simulink model "IEEE33_TR_TEMPORAL_RECOGNIZABILITY_MASTER"  (R2026b)
settings: Solver=ode23t  StopTime=0.2  MaxStep=1e-5
undefined symbols (not defined in the file): Three_PhaseBreaker_class, Three_PhaseSeriesRLCLoad_class, Three_PhaseSource_class, Three_PhaseV_IMeasuremen_class
libraries: ee_lib x146, nesl_utility x106, fl_lib x33, eeRmsMeasurement x2
(part 4 of 7)

== system IEEE33_TR_TEMPORAL_RECOGNIZABILITY_MASTER/Bus_15/Bus_15 ==
  Current and Voltage Sensor (Three-Phase) : ee_lib/Sensors & Transducers/Current and Voltage Sensor (Three-Phase)  port_option=ee.enum.threePhasePort.expanded  vMeasurementType=1  outputUnit=2  SRated=100000000 V*A  VRated=500000 V  I_specify=off  I_priority=None  I=[ 0 0 0 ] A  I_nominal_specify=off  I_nominal_value=1  I_nominal_unit=A  V_specify=off  V_priority=None  V=[ 0 0 0 ] V  V_nominal_specify=off  V_nominal_value=1  V_nominal_unit=V
  Igain : Gain  Gain=Three_PhaseV_IMeasuremen_class('phase-to-phase','yes','off','off','off',100000000,500000).objParamMappingDerived.NewDerivedParam.IG
  PS-Simulink Converter : nesl_utility/PS-Simulink Converter  PhysicalDomain=network_engine_domain  SubClassName=ps_output  LeftPortType=input  RightPortType=output  PseudoPeriodic=off  Frequencies=[]  VectorFormat=1-D array  Unit=1  AffineConversion=off
  PS-Simulink Converter1 : nesl_utility/PS-Simulink Converter  PhysicalDomain=network_engine_domain  SubClassName=ps_output  LeftPortType=input  RightPortType=output  PseudoPeriodic=off  Frequencies=[]  VectorFormat=1-D array  Unit=1  AffineConversion=off
  Vgain : Gain  Gain=Three_PhaseV_IMeasuremen_class('phase-to-phase','yes','off','off','off',100000000,500000).objParamMappingDerived.NewDerivedParam.VG
  A : PMIOPort  Side=Left
  B : PMIOPort  Port=2  Side=Left
  C : PMIOPort  Port=3  Side=Left
  a : PMIOPort  Port=4  Side=Right
  b : PMIOPort  Port=5  Side=Right
  c : PMIOPort  Port=6  Side=Right
  Vabc : Outport  VectorParamsAs1DForOutWhenUnconnected=off
  Iabc : Outport  Port=2  VectorParamsAs1DForOutWhenUnconnected=off
  wires:
  Igain/1 -> Iabc/1
  Vgain/1 -> Vabc/1
  PS-Simulink Converter1/1 -> Igain/1
  PS-Simulink Converter/1 -> Vgain/1
  connections:
  Current and Voltage Sensor (Three-Phase)/RConn1 -- PS-Simulink Converter/LConn1
  Current and Voltage Sensor (Three-Phase)/RConn2 -- PS-Simulink Converter1/LConn1
  Current and Voltage Sensor (Three-Phase)/RConn5 -- c/RConn1
  Current and Voltage Sensor (Three-Phase)/RConn4 -- b/RConn1
  Current and Voltage Sensor (Three-Phase)/RConn3 -- a/RConn1
  Current and Voltage Sensor (Three-Phase)/LConn3 -- C/RConn1
  Current and Voltage Sensor (Three-Phase)/LConn1 -- A/RConn1
  Current and Voltage Sensor (Three-Phase)/LConn2 -- B/RConn1

== system IEEE33_TR_TEMPORAL_RECOGNIZABILITY_MASTER/Bus_15/CB3-2 ==
  com : Inport
  Add : Sum
  Circuit Breaker : ee_lib/Switches & Breakers/Circuit Breaker (Three-Phase)  port_option=ee.enum.threePhasePort.expanded  control_port_option=ee.enum.controlport.ps  R_closed=0.01 Ohm  G_open=Three_PhaseBreaker_class('open',1000000,Inf,[0.0166666666666667 0.0833333333333333],'on').objParamMappingDerived.NewDerivedParam.G_open 1/Ohm  threshold=0.5 V  breaker_behavior=ee.enum.switches.breakerBehavior.zeroCrossingEnable  i_th=1e-8 A
  Data Type Conversion : DataTypeConversion  OutDataTypeStr=double  SaturateOnIntegerOverflow=off  RndMeth=Floor
  NOT : Logic  Operator=NOT  IconShape=distinctive  AllPortsSameDT=off  OutDataTypeStr=boolean
  Simulink-PS Converter : nesl_utility/Simulink-PS Converter  PhysicalDomain=network_engine_domain  SubClassName=ps_input  LeftPortType=input  RightPortType=output  PseudoPeriodic=off  Frequencies=[]  NoiseDistribution=none  NoiseParameters=[]  Unit=1  AffineConversion=off  FilteringAndDerivatives=provide  SimscapeFilterOrder=1  InputFilterTimeConstant=0.001  UdotUserProvided=0
  Step : Step  Time=1e-6  InitialValue=Three_PhaseBreaker_class('open',1000000,Inf,[0.0166666666666667 0.0833333333333333],'on').objParamMappingDerived.NewDerivedParam.StepInitialValue  FinalValue=0  SampleTime=0
  A : PMIOPort  Side=Left
  B : PMIOPort  Port=2  Side=Left
  C : PMIOPort  Port=3  Side=Left
  a : PMIOPort  Port=4  Side=Right
  b : PMIOPort  Port=5  Side=Right
  c : PMIOPort  Port=6  Side=Right
  wires:
  com/1 -> Add/1
  Add/1 -> NOT/1
  Step/1 -> Add/2
  Data Type Conversion/1 -> Simulink-PS Converter/1
  NOT/1 -> Data Type Conversion/1
  connections:
  Circuit Breaker/LConn1 -- Simulink-PS Converter/RConn1
  c/RConn1 -- Circuit Breaker/RConn3
  b/RConn1 -- Circuit Breaker/RConn2
  a/RConn1 -- Circuit Breaker/RConn1
  Circuit Breaker/LConn4 -- C/RConn1
  Circuit Breaker/LConn3 -- B/RConn1
  Circuit Breaker/LConn2 -- A/RConn1

== system IEEE33_TR_TEMPORAL_RECOGNIZABILITY_MASTER/Bus_15/VI Recorder18 ==
  Vrec : Inport
  Irec : Inport  Port=2
  tag scope: I14to15=global, V14to15=global
  wires:
  Vrec/1 -> [V14to15]
  Irec/1 -> [I14to15]

== system IEEE33_TR_TEMPORAL_RECOGNIZABILITY_MASTER/Bus_16/Bus Load 16 ==
  Electrical Reference : fl_lib/Electrical/Electrical Elements/Electrical Reference
  Wye-Connected Load : ee_lib/Passive/RLC Assemblies/Wye-Connected Load  port_option=ee.enum.threePhasePort.expanded  parameterization=2  component_structure=4  component_structure_PQ=4  R=1 Ohm  L=0.001 H  C=1e-6 F  VRated=11594.6483 V  FRated=60 Hz  P=60000 W  Qpos=20000 V*A  Qneg=Three_PhaseSeriesRLCLoad_class(0).objParamMappingDerived.NewDerivedParam.Qneg V*A  R_parasitic=1e-6 Ohm  G_parasitic=1e-6 1/Ohm  R_parasitic_PQ=1e-6 Ohm  G_parasitic_PQ=1e-6 1/Ohm  Vmag0=11594.6483 V  Vang0=0 deg  Freq0=60 Hz  IL_specify=on  IL_priority=High  IL=[ 0 0 0 ] A  IL_nominal_specify=off  IL_nominal_value=1  IL_nominal_unit=A  VC_specify=on  VC_priority=High  VC=[ 0 0 0 ] V  VC_nominal_specify=off  VC_nominal_value=1  VC_nominal_unit=V
  A : PMIOPort  Side=Left
  B : PMIOPort  Port=2  Side=Left
  C : PMIOPort  Port=3  Side=Left
  connections:
  Electrical Reference/LConn1 -- Wye-Connected Load/RConn1
  Wye-Connected Load/LConn3 -- C/RConn1
  Wye-Connected Load/LConn1 -- A/RConn1
  Wye-Connected Load/LConn2 -- B/RConn1

== system IEEE33_TR_TEMPORAL_RECOGNIZABILITY_MASTER/Bus_16/Bus_16 ==
  Current and Voltage Sensor (Three-Phase) : ee_lib/Sensors & Transducers/Current and Voltage Sensor (Three-Phase)  port_option=ee.enum.threePhasePort.expanded  vMeasurementType=1  outputUnit=2  SRated=100000000 V*A  VRated=500000 V  I_specify=off  I_priority=None  I=[ 0 0 0 ] A  I_nominal_specify=off  I_nominal_value=1  I_nominal_unit=A  V_specify=off  V_priority=None  V=[ 0 0 0 ] V  V_nominal_specify=off  V_nominal_value=1  V_nominal_unit=V
  Igain : Gain  Gain=Three_PhaseV_IMeasuremen_class('phase-to-phase','yes','off','off','off',100000000,500000).objParamMappingDerived.NewDerivedParam.IG
  PS-Simulink Converter : nesl_utility/PS-Simulink Converter  PhysicalDomain=network_engine_domain  SubClassName=ps_output  LeftPortType=input  RightPortType=output  PseudoPeriodic=off  Frequencies=[]  VectorFormat=1-D array  Unit=1  AffineConversion=off
  PS-Simulink Converter1 : nesl_utility/PS-Simulink Converter  PhysicalDomain=network_engine_domain  SubClassName=ps_output  LeftPortType=input  RightPortType=output  PseudoPeriodic=off  Frequencies=[]  VectorFormat=1-D array  Unit=1  AffineConversion=off
  Vgain : Gain  Gain=Three_PhaseV_IMeasuremen_class('phase-to-phase','yes','off','off','off',100000000,500000).objParamMappingDerived.NewDerivedParam.VG
  A : PMIOPort  Side=Left
  B : PMIOPort  Port=2  Side=Left
  C : PMIOPort  Port=3  Side=Left
  a : PMIOPort  Port=4  Side=Right
  b : PMIOPort  Port=5  Side=Right
  c : PMIOPort  Port=6  Side=Right
  Vabc : Outport  VectorParamsAs1DForOutWhenUnconnected=off
  Iabc : Outport  Port=2  VectorParamsAs1DForOutWhenUnconnected=off
  wires:
  Igain/1 -> Iabc/1
  Vgain/1 -> Vabc/1
  PS-Simulink Converter1/1 -> Igain/1
  PS-Simulink Converter/1 -> Vgain/1
  connections:
  Current and Voltage Sensor (Three-Phase)/RConn1 -- PS-Simulink Converter/LConn1
  Current and Voltage Sensor (Three-Phase)/RConn2 -- PS-Simulink Converter1/LConn1
  Current and Voltage Sensor (Three-Phase)/RConn5 -- c/RConn1
  Current and Voltage Sensor (Three-Phase)/RConn4 -- b/RConn1
  Current and Voltage Sensor (Three-Phase)/RConn3 -- a/RConn1
  Current and Voltage Sensor (Three-Phase)/LConn3 -- C/RConn1
  Current and Voltage Sensor (Three-Phase)/LConn1 -- A/RConn1
  Current and Voltage Sensor (Three-Phase)/LConn2 -- B/RConn1

== system IEEE33_TR_TEMPORAL_RECOGNIZABILITY_MASTER/Bus_16/CB3-2 ==
  com : Inport
  Add : Sum
  Circuit Breaker : ee_lib/Switches & Breakers/Circuit Breaker (Three-Phase)  port_option=ee.enum.threePhasePort.expanded  control_port_option=ee.enum.controlport.ps  R_closed=0.01 Ohm  G_open=Three_PhaseBreaker_class('open',1000000,Inf,[0.0166666666666667 0.0833333333333333],'on').objParamMappingDerived.NewDerivedParam.G_open 1/Ohm  threshold=0.5 V  breaker_behavior=ee.enum.switches.breakerBehavior.zeroCrossingEnable  i_th=1e-8 A
  Data Type Conversion : DataTypeConversion  OutDataTypeStr=double  SaturateOnIntegerOverflow=off  RndMeth=Floor
  NOT : Logic  Operator=NOT  IconShape=distinctive  AllPortsSameDT=off  OutDataTypeStr=boolean
  Simulink-PS Converter : nesl_utility/Simulink-PS Converter  PhysicalDomain=network_engine_domain  SubClassName=ps_input  LeftPortType=input  RightPortType=output  PseudoPeriodic=off  Frequencies=[]  NoiseDistribution=none  NoiseParameters=[]  Unit=1  AffineConversion=off  FilteringAndDerivatives=provide  SimscapeFilterOrder=1  InputFilterTimeConstant=0.001  UdotUserProvided=0
  Step : Step  Time=1e-6  InitialValue=Three_PhaseBreaker_class('open',1000000,Inf,[0.0166666666666667 0.0833333333333333],'on').objParamMappingDerived.NewDerivedParam.StepInitialValue  FinalValue=0  SampleTime=0
  A : PMIOPort  Side=Left
  B : PMIOPort  Port=2  Side=Left
  C : PMIOPort  Port=3  Side=Left
  a : PMIOPort  Port=4  Side=Right
  b : PMIOPort  Port=5  Side=Right
  c : PMIOPort  Port=6  Side=Right
  wires:
  com/1 -> Add/1
  Add/1 -> NOT/1
  Step/1 -> Add/2
  Data Type Conversion/1 -> Simulink-PS Converter/1
  NOT/1 -> Data Type Conversion/1
  connections:
  Circuit Breaker/LConn1 -- Simulink-PS Converter/RConn1
  c/RConn1 -- Circuit Breaker/RConn3
  b/RConn1 -- Circuit Breaker/RConn2
  a/RConn1 -- Circuit Breaker/RConn1
  Circuit Breaker/LConn4 -- C/RConn1
  Circuit Breaker/LConn3 -- B/RConn1
  Circuit Breaker/LConn2 -- A/RConn1

== system IEEE33_TR_TEMPORAL_RECOGNIZABILITY_MASTER/Bus_16/VI Recorder19 ==
  Vrec : Inport
  Irec : Inport  Port=2
  tag scope: I15to16=global, V15to16=global
  wires:
  Vrec/1 -> [V15to16]
  Irec/1 -> [I15to16]

== system IEEE33_TR_TEMPORAL_RECOGNIZABILITY_MASTER/Bus_17/Bus Load 17 ==
  Electrical Reference : fl_lib/Electrical/Electrical Elements/Electrical Reference
  Wye-Connected Load : ee_lib/Passive/RLC Assemblies/Wye-Connected Load  port_option=ee.enum.threePhasePort.expanded  parameterization=2  component_structure=4  component_structure_PQ=4  R=1 Ohm  L=0.001 H  C=1e-6 F  VRated=11569.0372 V  FRated=60 Hz  P=60000 W  Qpos=20000 V*A  Qneg=Three_PhaseSeriesRLCLoad_class(0).objParamMappingDerived.NewDerivedParam.Qneg V*A  R_parasitic=1e-6 Ohm  G_parasitic=1e-6 1/Ohm  R_parasitic_PQ=1e-6 Ohm  G_parasitic_PQ=1e-6 1/Ohm  Vmag0=11569.0372 V  Vang0=0 deg  Freq0=60 Hz  IL_specify=on  IL_priority=High  IL=[ 0 0 0 ] A  IL_nominal_specify=off  IL_nominal_value=1  IL_nominal_unit=A  VC_specify=on  VC_priority=High  VC=[ 0 0 0 ] V  VC_nominal_specify=off  VC_nominal_value=1  VC_nominal_unit=V
  A : PMIOPort  Side=Left
  B : PMIOPort  Port=2  Side=Left
  C : PMIOPort  Port=3  Side=Left
  connections:
  Electrical Reference/LConn1 -- Wye-Connected Load/RConn1
  Wye-Connected Load/LConn3 -- C/RConn1
  Wye-Connected Load/LConn1 -- A/RConn1
  Wye-Connected Load/LConn2 -- B/RConn1

== system IEEE33_TR_TEMPORAL_RECOGNIZABILITY_MASTER/Bus_17/Bus_17 ==
  Current and Voltage Sensor (Three-Phase) : ee_lib/Sensors & Transducers/Current and Voltage Sensor (Three-Phase)  port_option=ee.enum.threePhasePort.expanded  vMeasurementType=1  outputUnit=2  SRated=100000000 V*A  VRated=500000 V  I_specify=off  I_priority=None  I=[ 0 0 0 ] A  I_nominal_specify=off  I_nominal_value=1  I_nominal_unit=A  V_specify=off  V_priority=None  V=[ 0 0 0 ] V  V_nominal_specify=off  V_nominal_value=1  V_nominal_unit=V
  Igain : Gain  Gain=Three_PhaseV_IMeasuremen_class('phase-to-phase','yes','off','off','off',100000000,500000).objParamMappingDerived.NewDerivedParam.IG
  PS-Simulink Converter : nesl_utility/PS-Simulink Converter  PhysicalDomain=network_engine_domain  SubClassName=ps_output  LeftPortType=input  RightPortType=output  PseudoPeriodic=off  Frequencies=[]  VectorFormat=1-D array  Unit=1  AffineConversion=off
  PS-Simulink Converter1 : nesl_utility/PS-Simulink Converter  PhysicalDomain=network_engine_domain  SubClassName=ps_output  LeftPortType=input  RightPortType=output  PseudoPeriodic=off  Frequencies=[]  VectorFormat=1-D array  Unit=1  AffineConversion=off
  Vgain : Gain  Gain=Three_PhaseV_IMeasuremen_class('phase-to-phase','yes','off','off','off',100000000,500000).objParamMappingDerived.NewDerivedParam.VG
  A : PMIOPort  Side=Left
  B : PMIOPort  Port=2  Side=Left
  C : PMIOPort  Port=3  Side=Left
  a : PMIOPort  Port=4  Side=Right
  b : PMIOPort  Port=5  Side=Right
  c : PMIOPort  Port=6  Side=Right
  Vabc : Outport  VectorParamsAs1DForOutWhenUnconnected=off
  Iabc : Outport  Port=2  VectorParamsAs1DForOutWhenUnconnected=off
  wires:
  Igain/1 -> Iabc/1
  Vgain/1 -> Vabc/1
  PS-Simulink Converter1/1 -> Igain/1
  PS-Simulink Converter/1 -> Vgain/1
  connections:
  Current and Voltage Sensor (Three-Phase)/RConn1 -- PS-Simulink Converter/LConn1
  Current and Voltage Sensor (Three-Phase)/RConn2 -- PS-Simulink Converter1/LConn1
  Current and Voltage Sensor (Three-Phase)/RConn5 -- c/RConn1
  Current and Voltage Sensor (Three-Phase)/RConn4 -- b/RConn1
  Current and Voltage Sensor (Three-Phase)/RConn3 -- a/RConn1
  Current and Voltage Sensor (Three-Phase)/LConn3 -- C/RConn1
  Current and Voltage Sensor (Three-Phase)/LConn1 -- A/RConn1
  Current and Voltage Sensor (Three-Phase)/LConn2 -- B/RConn1

== system IEEE33_TR_TEMPORAL_RECOGNIZABILITY_MASTER/Bus_17/CB3-2 ==
  com : Inport
  Add : Sum
  Circuit Breaker : ee_lib/Switches & Breakers/Circuit Breaker (Three-Phase)  port_option=ee.enum.threePhasePort.expanded  control_port_option=ee.enum.controlport.ps  R_closed=0.01 Ohm  G_open=Three_PhaseBreaker_class('open',1000000,Inf,[0.0166666666666667 0.0833333333333333],'on').objParamMappingDerived.NewDerivedParam.G_open 1/Ohm  threshold=0.5 V  breaker_behavior=ee.enum.switches.breakerBehavior.zeroCrossingEnable  i_th=1e-8 A
  Data Type Conversion : DataTypeConversion  OutDataTypeStr=double  SaturateOnIntegerOverflow=off  RndMeth=Floor
  NOT : Logic  Operator=NOT  IconShape=distinctive  AllPortsSameDT=off  OutDataTypeStr=boolean
  Simulink-PS Converter : nesl_utility/Simulink-PS Converter  PhysicalDomain=network_engine_domain  SubClassName=ps_input  LeftPortType=input  RightPortType=output  PseudoPeriodic=off  Frequencies=[]  NoiseDistribution=none  NoiseParameters=[]  Unit=1  AffineConversion=off  FilteringAndDerivatives=provide  SimscapeFilterOrder=1  InputFilterTimeConstant=0.001  UdotUserProvided=0
  Step : Step  Time=1e-6  InitialValue=Three_PhaseBreaker_class('open',1000000,Inf,[0.0166666666666667 0.0833333333333333],'on').objParamMappingDerived.NewDerivedParam.StepInitialValue  FinalValue=0  SampleTime=0
  A : PMIOPort  Side=Left
  B : PMIOPort  Port=2  Side=Left
  C : PMIOPort  Port=3  Side=Left
  a : PMIOPort  Port=4  Side=Right
  b : PMIOPort  Port=5  Side=Right
  c : PMIOPort  Port=6  Side=Right
  wires:
  com/1 -> Add/1
  Add/1 -> NOT/1
  Step/1 -> Add/2
  Data Type Conversion/1 -> Simulink-PS Converter/1
  NOT/1 -> Data Type Conversion/1
  connections:
  Circuit Breaker/LConn1 -- Simulink-PS Converter/RConn1
  c/RConn1 -- Circuit Breaker/RConn3
  b/RConn1 -- Circuit Breaker/RConn2
  a/RConn1 -- Circuit Breaker/RConn1
  Circuit Breaker/LConn4 -- C/RConn1
  Circuit Breaker/LConn3 -- B/RConn1
  Circuit Breaker/LConn2 -- A/RConn1

== system IEEE33_TR_TEMPORAL_RECOGNIZABILITY_MASTER/Bus_17/VI Recorder20 ==
  Vrec : Inport
  Irec : Inport  Port=2
  tag scope: I16to17=global, V16to17=global
  wires:
  Vrec/1 -> [V16to17]
  Irec/1 -> [I16to17]

== system IEEE33_TR_TEMPORAL_RECOGNIZABILITY_MASTER/Bus_18/Bus Load 18 ==
  Electrical Reference : fl_lib/Electrical/Electrical Elements/Electrical Reference
  Wye-Connected Load : ee_lib/Passive/RLC Assemblies/Wye-Connected Load  port_option=ee.enum.threePhasePort.expanded  parameterization=2  component_structure=4  component_structure_PQ=4  R=1 Ohm  L=0.001 H  C=1e-6 F  VRated=11561.3652 V  FRated=60 Hz  P=90000 W  Qpos=40000 V*A  Qneg=Three_PhaseSeriesRLCLoad_class(0).objParamMappingDerived.NewDerivedParam.Qneg V*A  R_parasitic=1e-6 Ohm  G_parasitic=1e-6 1/Ohm  R_parasitic_PQ=1e-6 Ohm  G_parasitic_PQ=1e-6 1/Ohm  Vmag0=11561.3652 V  Vang0=0 deg  Freq0=60 Hz  IL_specify=on  IL_priority=High  IL=[ 0 0 0 ] A  IL_nominal_specify=off  IL_nominal_value=1  IL_nominal_unit=A  VC_specify=on  VC_priority=High  VC=[ 0 0 0 ] V  VC_nominal_specify=off  VC_nominal_value=1  VC_nominal_unit=V
  A : PMIOPort  Side=Left
  B : PMIOPort  Port=2  Side=Left
  C : PMIOPort  Port=3  Side=Left
  connections:
  Electrical Reference/LConn1 -- Wye-Connected Load/RConn1
  Wye-Connected Load/LConn3 -- C/RConn1
  Wye-Connected Load/LConn1 -- A/RConn1
  Wye-Connected Load/LConn2 -- B/RConn1

== system IEEE33_TR_TEMPORAL_RECOGNIZABILITY_MASTER/Bus_18/Bus_18 ==
  Current and Voltage Sensor (Three-Phase) : ee_lib/Sensors & Transducers/Current and Voltage Sensor (Three-Phase)  port_option=ee.enum.threePhasePort.expanded  vMeasurementType=1  outputUnit=2  SRated=100000000 V*A  VRated=500000 V  I_specify=off  I_priority=None  I=[ 0 0 0 ] A  I_nominal_specify=off  I_nominal_value=1  I_nominal_unit=A  V_specify=off  V_priority=None  V=[ 0 0 0 ] V  V_nominal_specify=off  V_nominal_value=1  V_nominal_unit=V
  Igain : Gain  Gain=Three_PhaseV_IMeasuremen_class('phase-to-phase','yes','off','off','off',100000000,500000).objParamMappingDerived.NewDerivedParam.IG
  PS-Simulink Converter : nesl_utility/PS-Simulink Converter  PhysicalDomain=network_engine_domain  SubClassName=ps_output  LeftPortType=input  RightPortType=output  PseudoPeriodic=off  Frequencies=[]  VectorFormat=1-D array  Unit=1  AffineConversion=off
  PS-Simulink Converter1 : nesl_utility/PS-Simulink Converter  PhysicalDomain=network_engine_domain  SubClassName=ps_output  LeftPortType=input  RightPortType=output  PseudoPeriodic=off  Frequencies=[]  VectorFormat=1-D array  Unit=1  AffineConversion=off
  Vgain : Gain  Gain=Three_PhaseV_IMeasuremen_class('phase-to-phase','yes','off','off','off',100000000,500000).objParamMappingDerived.NewDerivedParam.VG
  A : PMIOPort  Side=Left
  B : PMIOPort  Port=2  Side=Left
  C : PMIOPort  Port=3  Side=Left
  a : PMIOPort  Port=4  Side=Right
  b : PMIOPort  Port=5  Side=Right
  c : PMIOPort  Port=6  Side=Right
  Vabc : Outport  VectorParamsAs1DForOutWhenUnconnected=off
  Iabc : Outport  Port=2  VectorParamsAs1DForOutWhenUnconnected=off
  wires:
  Igain/1 -> Iabc/1
  Vgain/1 -> Vabc/1
  PS-Simulink Converter1/1 -> Igain/1
  PS-Simulink Converter/1 -> Vgain/1
  connections:
  Current and Voltage Sensor (Three-Phase)/RConn1 -- PS-Simulink Converter/LConn1
  Current and Voltage Sensor (Three-Phase)/RConn2 -- PS-Simulink Converter1/LConn1
  Current and Voltage Sensor (Three-Phase)/RConn5 -- c/RConn1
  Current and Voltage Sensor (Three-Phase)/RConn4 -- b/RConn1
  Current and Voltage Sensor (Three-Phase)/RConn3 -- a/RConn1
  Current and Voltage Sensor (Three-Phase)/LConn3 -- C/RConn1
  Current and Voltage Sensor (Three-Phase)/LConn1 -- A/RConn1
  Current and Voltage Sensor (Three-Phase)/LConn2 -- B/RConn1

== system IEEE33_TR_TEMPORAL_RECOGNIZABILITY_MASTER/Bus_18/CB3-2 ==
  com : Inport
  Add : Sum
  Circuit Breaker : ee_lib/Switches & Breakers/Circuit Breaker (Three-Phase)  port_option=ee.enum.threePhasePort.expanded  control_port_option=ee.enum.controlport.ps  R_closed=0.01 Ohm  G_open=Three_PhaseBreaker_class('open',1000000,Inf,[0.0166666666666667 0.0833333333333333],'on').objParamMappingDerived.NewDerivedParam.G_open 1/Ohm  threshold=0.5 V  breaker_behavior=ee.enum.switches.breakerBehavior.zeroCrossingEnable  i_th=1e-8 A
  Data Type Conversion : DataTypeConversion  OutDataTypeStr=double  SaturateOnIntegerOverflow=off  RndMeth=Floor
  NOT : Logic  Operator=NOT  IconShape=distinctive  AllPortsSameDT=off  OutDataTypeStr=boolean
  Simulink-PS Converter : nesl_utility/Simulink-PS Converter  PhysicalDomain=network_engine_domain  SubClassName=ps_input  LeftPortType=input  RightPortType=output  PseudoPeriodic=off  Frequencies=[]  NoiseDistribution=none  NoiseParameters=[]  Unit=1  AffineConversion=off  FilteringAndDerivatives=provide  SimscapeFilterOrder=1  InputFilterTimeConstant=0.001  UdotUserProvided=0
  Step : Step  Time=1e-6  InitialValue=Three_PhaseBreaker_class('open',1000000,Inf,[0.0166666666666667 0.0833333333333333],'on').objParamMappingDerived.NewDerivedParam.StepInitialValue  FinalValue=0  SampleTime=0
  A : PMIOPort  Side=Left
  B : PMIOPort  Port=2  Side=Left
  C : PMIOPort  Port=3  Side=Left
  a : PMIOPort  Port=4  Side=Right
  b : PMIOPort  Port=5  Side=Right
  c : PMIOPort  Port=6  Side=Right
  wires:
  com/1 -> Add/1
  Add/1 -> NOT/1
  Step/1 -> Add/2
  Data Type Conversion/1 -> Simulink-PS Converter/1
  NOT/1 -> Data Type Conversion/1
  connections:
  Circuit Breaker/LConn1 -- Simulink-PS Converter/RConn1
  c/RConn1 -- Circuit Breaker/RConn3
  b/RConn1 -- Circuit Breaker/RConn2
  a/RConn1 -- Circuit Breaker/RConn1
  Circuit Breaker/LConn4 -- C/RConn1
  Circuit Breaker/LConn3 -- B/RConn1
  Circuit Breaker/LConn2 -- A/RConn1

== system IEEE33_TR_TEMPORAL_RECOGNIZABILITY_MASTER/Bus_18/VI Recorder21 ==
  Vrec : Inport
  Irec : Inport  Port=2
  tag scope: I17to18=global, V17to18=global
  wires:
  Vrec/1 -> [V17to18]
  Irec/1 -> [I17to18]

== system IEEE33_TR_TEMPORAL_RECOGNIZABILITY_MASTER/Bus_19/Bus Load 19 ==
  Electrical Reference : fl_lib/Electrical/Electrical Elements/Electrical Reference
  Wye-Connected Load : ee_lib/Passive/RLC Assemblies/Wye-Connected Load  port_option=ee.enum.threePhasePort.expanded  parameterization=2  component_structure=4  component_structure_PQ=4  R=1 Ohm  L=0.001 H  C=1e-6 F  VRated=12615.7786 V  FRated=60 Hz  P=90000 W  Qpos=40000 V*A  Qneg=Three_PhaseSeriesRLCLoad_class(0).objParamMappingDerived.NewDerivedParam.Qneg V*A  R_parasitic=1e-6 Ohm  G_parasitic=1e-6 1/Ohm  R_parasitic_PQ=1e-6 Ohm  G_parasitic_PQ=1e-6 1/Ohm  Vmag0=12615.7786 V  Vang0=0 deg  Freq0=60 Hz  IL_specify=on  IL_priority=High  IL=[ 0 0 0 ] A  IL_nominal_specify=off  IL_nominal_value=1  IL_nominal_unit=A  VC_specify=on  VC_priority=High  VC=[ 0 0 0 ] V  VC_nominal_specify=off  VC_nominal_value=1  VC_nominal_unit=V
  A : PMIOPort  Side=Left
  B : PMIOPort  Port=2  Side=Left
  C : PMIOPort  Port=3  Side=Left
  connections:
  Electrical Reference/LConn1 -- Wye-Connected Load/RConn1
  Wye-Connected Load/LConn3 -- C/RConn1
  Wye-Connected Load/LConn1 -- A/RConn1
  Wye-Connected Load/LConn2 -- B/RConn1

== system IEEE33_TR_TEMPORAL_RECOGNIZABILITY_MASTER/Bus_19/Bus_19 ==
  Current and Voltage Sensor (Three-Phase) : ee_lib/Sensors & Transducers/Current and Voltage Sensor (Three-Phase)  port_option=ee.enum.threePhasePort.expanded  vMeasurementType=1  outputUnit=2  SRated=100000000 V*A  VRated=500000 V  I_specify=off  I_priority=None  I=[ 0 0 0 ] A  I_nominal_specify=off  I_nominal_value=1  I_nominal_unit=A  V_specify=off  V_priority=None  V=[ 0 0 0 ] V  V_nominal_specify=off  V_nominal_value=1  V_nominal_unit=V
  Igain : Gain  Gain=Three_PhaseV_IMeasuremen_class('phase-to-phase','yes','off','off','off',100000000,500000).objParamMappingDerived.NewDerivedParam.IG
  PS-Simulink Converter : nesl_utility/PS-Simulink Converter  PhysicalDomain=network_engine_domain  SubClassName=ps_output  LeftPortType=input  RightPortType=output  PseudoPeriodic=off  Frequencies=[]  VectorFormat=1-D array  Unit=1  AffineConversion=off
  PS-Simulink Converter1 : nesl_utility/PS-Simulink Converter  PhysicalDomain=network_engine_domain  SubClassName=ps_output  LeftPortType=input  RightPortType=output  PseudoPeriodic=off  Frequencies=[]  VectorFormat=1-D array  Unit=1  AffineConversion=off
  Vgain : Gain  Gain=Three_PhaseV_IMeasuremen_class('phase-to-phase','yes','off','off','off',100000000,500000).objParamMappingDerived.NewDerivedParam.VG
  A : PMIOPort  Side=Left
  B : PMIOPort  Port=2  Side=Left
  C : PMIOPort  Port=3  Side=Left
  a : PMIOPort  Port=4  Side=Right
  b : PMIOPort  Port=5  Side=Right
  c : PMIOPort  Port=6  Side=Right
  Vabc : Outport  VectorParamsAs1DForOutWhenUnconnected=off
  Iabc : Outport  Port=2  VectorParamsAs1DForOutWhenUnconnected=off
  wires:
  Igain/1 -> Iabc/1
  Vgain/1 -> Vabc/1
  PS-Simulink Converter1/1 -> Igain/1
  PS-Simulink Converter/1 -> Vgain/1
  connections:
  Current and Voltage Sensor (Three-Phase)/RConn1 -- PS-Simulink Converter/LConn1
  Current and Voltage Sensor (Three-Phase)/RConn2 -- PS-Simulink Converter1/LConn1
  Current and Voltage Sensor (Three-Phase)/RConn5 -- c/RConn1
  Current and Voltage Sensor (Three-Phase)/RConn4 -- b/RConn1
  Current and Voltage Sensor (Three-Phase)/RConn3 -- a/RConn1
  Current and Voltage Sensor (Three-Phase)/LConn3 -- C/RConn1
  Current and Voltage Sensor (Three-Phase)/LConn1 -- A/RConn1
  Current and Voltage Sensor (Three-Phase)/LConn2 -- B/RConn1

== system IEEE33_TR_TEMPORAL_RECOGNIZABILITY_MASTER/Bus_19/CB3-2 ==
  com : Inport
  Add : Sum
  Circuit Breaker : ee_lib/Switches & Breakers/Circuit Breaker (Three-Phase)  port_option=ee.enum.threePhasePort.expanded  control_port_option=ee.enum.controlport.ps  R_closed=0.01 Ohm  G_open=Three_PhaseBreaker_class('open',1000000,Inf,[0.0166666666666667 0.0833333333333333],'on').objParamMappingDerived.NewDerivedParam.G_open 1/Ohm  threshold=0.5 V  breaker_behavior=ee.enum.switches.breakerBehavior.zeroCrossingEnable  i_th=1e-8 A
  Data Type Conversion : DataTypeConversion  OutDataTypeStr=double  SaturateOnIntegerOverflow=off  RndMeth=Floor
  NOT : Logic  Operator=NOT  IconShape=distinctive  AllPortsSameDT=off  OutDataTypeStr=boolean
  Simulink-PS Converter : nesl_utility/Simulink-PS Converter  PhysicalDomain=network_engine_domain  SubClassName=ps_input  LeftPortType=input  RightPortType=output  PseudoPeriodic=off  Frequencies=[]  NoiseDistribution=none  NoiseParameters=[]  Unit=1  AffineConversion=off  FilteringAndDerivatives=provide  SimscapeFilterOrder=1  InputFilterTimeConstant=0.001  UdotUserProvided=0
  Step : Step  Time=1e-6  InitialValue=Three_PhaseBreaker_class('open',1000000,Inf,[0.0166666666666667 0.0833333333333333],'on').objParamMappingDerived.NewDerivedParam.StepInitialValue  FinalValue=0  SampleTime=0
  A : PMIOPort  Side=Left
  B : PMIOPort  Port=2  Side=Left
  C : PMIOPort  Port=3  Side=Left
  a : PMIOPort  Port=4  Side=Right
  b : PMIOPort  Port=5  Side=Right
  c : PMIOPort  Port=6  Side=Right
  wires:
  com/1 -> Add/1
  Add/1 -> NOT/1
  Step/1 -> Add/2
  Data Type Conversion/1 -> Simulink-PS Converter/1
  NOT/1 -> Data Type Conversion/1
  connections:
  Circuit Breaker/LConn1 -- Simulink-PS Converter/RConn1
  c/RConn1 -- Circuit Breaker/RConn3
  b/RConn1 -- Circuit Breaker/RConn2
  a/RConn1 -- Circuit Breaker/RConn1
  Circuit Breaker/LConn4 -- C/RConn1
  Circuit Breaker/LConn3 -- B/RConn1
  Circuit Breaker/LConn2 -- A/RConn1

== system IEEE33_TR_TEMPORAL_RECOGNIZABILITY_MASTER/Bus_19/VI Recorder ==
  Vrec : Inport
  Irec : Inport  Port=2
  tag scope: I2to19=global, V2to19=global
  wires:
  Vrec/1 -> [V2to19]
  Irec/1 -> [I2to19]

== system IEEE33_TR_TEMPORAL_RECOGNIZABILITY_MASTER/Bus_2/Bus Load 2 ==
  Electrical Reference : fl_lib/Electrical/Electrical Elements/Electrical Reference
  Wye-Connected Load : ee_lib/Passive/RLC Assemblies/Wye-Connected Load  port_option=ee.enum.threePhasePort.expanded  parameterization=2  component_structure=4  component_structure_PQ=4  R=1 Ohm  L=0.001 H  C=1e-6 F  VRated=12622.4631 V  FRated=60 Hz  P=100000 W  Qpos=60000 V*A  Qneg=Three_PhaseSeriesRLCLoad_class(0).objParamMappingDerived.NewDerivedParam.Qneg V*A  R_parasitic=1e-6 Ohm  G_parasitic=1e-6 1/Ohm  R_parasitic_PQ=1e-6 Ohm  G_parasitic_PQ=1e-6 1/Ohm  Vmag0=12622.4631 V  Vang0=0 deg  Freq0=60 Hz  IL_specify=on  IL_priority=High  IL=[ 0 0 0 ] A  IL_nominal_specify=off  IL_nominal_value=1  IL_nominal_unit=A  VC_specify=on  VC_priority=High  VC=[ 0 0 0 ] V  VC_nominal_specify=off  VC_nominal_value=1  VC_nominal_unit=V
  A : PMIOPort  Side=Left
  B : PMIOPort  Port=2  Side=Left
  C : PMIOPort  Port=3  Side=Left
  connections:
  Electrical Reference/LConn1 -- Wye-Connected Load/RConn1
  Wye-Connected Load/LConn3 -- C/RConn1
  Wye-Connected Load/LConn1 -- A/RConn1
  Wye-Connected Load/LConn2 -- B/RConn1

== system IEEE33_TR_TEMPORAL_RECOGNIZABILITY_MASTER/Bus_2/Bus_2 ==
  Current and Voltage Sensor (Three-Phase) : ee_lib/Sensors & Transducers/Current and Voltage Sensor (Three-Phase)  port_option=ee.enum.threePhasePort.expanded  vMeasurementType=1  outputUnit=2  SRated=100000000 V*A  VRated=500000 V  I_specify=off  I_priority=None  I=[ 0 0 0 ] A  I_nominal_specify=off  I_nominal_value=1  I_nominal_unit=A  V_specify=off  V_priority=None  V=[ 0 0 0 ] V  V_nominal_specify=off  V_nominal_value=1  V_nominal_unit=V
  Igain : Gain  Gain=Three_PhaseV_IMeasuremen_class('phase-to-phase','yes','off','off','off',100000000,500000).objParamMappingDerived.NewDerivedParam.IG
  PS-Simulink Converter : nesl_utility/PS-Simulink Converter  PhysicalDomain=network_engine_domain  SubClassName=ps_output  LeftPortType=input  RightPortType=output  PseudoPeriodic=off  Frequencies=[]  VectorFormat=1-D array  Unit=1  AffineConversion=off
  PS-Simulink Converter1 : nesl_utility/PS-Simulink Converter  PhysicalDomain=network_engine_domain  SubClassName=ps_output  LeftPortType=input  RightPortType=output  PseudoPeriodic=off  Frequencies=[]  VectorFormat=1-D array  Unit=1  AffineConversion=off
  Vgain : Gain  Gain=Three_PhaseV_IMeasuremen_class('phase-to-phase','yes','off','off','off',100000000,500000).objParamMappingDerived.NewDerivedParam.VG
  A : PMIOPort  Side=Left
  B : PMIOPort  Port=2  Side=Left
  C : PMIOPort  Port=3  Side=Left
  a : PMIOPort  Port=4  Side=Right
  b : PMIOPort  Port=5  Side=Right
  c : PMIOPort  Port=6  Side=Right
  Vabc : Outport  VectorParamsAs1DForOutWhenUnconnected=off
  Iabc : Outport  Port=2  VectorParamsAs1DForOutWhenUnconnected=off
  wires:
  Igain/1 -> Iabc/1
  Vgain/1 -> Vabc/1
  PS-Simulink Converter1/1 -> Igain/1
  PS-Simulink Converter/1 -> Vgain/1
  connections:
  Current and Voltage Sensor (Three-Phase)/RConn1 -- PS-Simulink Converter/LConn1
  Current and Voltage Sensor (Three-Phase)/RConn2 -- PS-Simulink Converter1/LConn1
  Current and Voltage Sensor (Three-Phase)/RConn5 -- c/RConn1
  Current and Voltage Sensor (Three-Phase)/RConn4 -- b/RConn1
  Current and Voltage Sensor (Three-Phase)/RConn3 -- a/RConn1
  Current and Voltage Sensor (Three-Phase)/LConn3 -- C/RConn1
  Current and Voltage Sensor (Three-Phase)/LConn1 -- A/RConn1
  Current and Voltage Sensor (Three-Phase)/LConn2 -- B/RConn1

== system IEEE33_TR_TEMPORAL_RECOGNIZABILITY_MASTER/Bus_2/CB3-1 ==
  com : Inport
  Add : Sum
  Circuit Breaker : ee_lib/Switches & Breakers/Circuit Breaker (Three-Phase)  port_option=ee.enum.threePhasePort.expanded  control_port_option=ee.enum.controlport.ps  R_closed=0.01 Ohm  G_open=Three_PhaseBreaker_class('open',1000000,Inf,[0.0166666666666667 0.0833333333333333],'on').objParamMappingDerived.NewDerivedParam.G_open 1/Ohm  threshold=0.5 V  breaker_behavior=ee.enum.switches.breakerBehavior.zeroCrossingEnable  i_th=1e-8 A
  Data Type Conversion : DataTypeConversion  OutDataTypeStr=double  SaturateOnIntegerOverflow=off  RndMeth=Floor
  NOT : Logic  Operator=NOT  IconShape=distinctive  AllPortsSameDT=off  OutDataTypeStr=boolean
  Simulink-PS Converter : nesl_utility/Simulink-PS Converter  PhysicalDomain=network_engine_domain  SubClassName=ps_input  LeftPortType=input  RightPortType=output  PseudoPeriodic=off  Frequencies=[]  NoiseDistribution=none  NoiseParameters=[]  Unit=1  AffineConversion=off  FilteringAndDerivatives=provide  SimscapeFilterOrder=1  InputFilterTimeConstant=0.001  UdotUserProvided=0
  Step : Step  Time=1e-6  InitialValue=Three_PhaseBreaker_class('open',1000000,Inf,[0.0166666666666667 0.0833333333333333],'on').objParamMappingDerived.NewDerivedParam.StepInitialValue  FinalValue=0  SampleTime=0
  A : PMIOPort  Side=Left
  B : PMIOPort  Port=2  Side=Left
  C : PMIOPort  Port=3  Side=Left
  a : PMIOPort  Port=4  Side=Right
  b : PMIOPort  Port=5  Side=Right
  c : PMIOPort  Port=6  Side=Right
  wires:
  com/1 -> Add/1
  Add/1 -> NOT/1
  Step/1 -> Add/2
  Data Type Conversion/1 -> Simulink-PS Converter/1
  NOT/1 -> Data Type Conversion/1
  connections:
  Circuit Breaker/LConn1 -- Simulink-PS Converter/RConn1
  c/RConn1 -- Circuit Breaker/RConn3
  b/RConn1 -- Circuit Breaker/RConn2
  a/RConn1 -- Circuit Breaker/RConn1
  Circuit Breaker/LConn4 -- C/RConn1
  Circuit Breaker/LConn3 -- B/RConn1
  Circuit Breaker/LConn2 -- A/RConn1

== system IEEE33_TR_TEMPORAL_RECOGNIZABILITY_MASTER/Bus_2/CB3-2 ==
  com : Inport
  Add : Sum
  Circuit Breaker : ee_lib/Switches & Breakers/Circuit Breaker (Three-Phase)  port_option=ee.enum.threePhasePort.expanded  control_port_option=ee.enum.controlport.ps  R_closed=0.01 Ohm  G_open=Three_PhaseBreaker_class('open',1000000,Inf,[0.0166666666666667 0.0833333333333333],'on').objParamMappingDerived.NewDerivedParam.G_open 1/Ohm  threshold=0.5 V  breaker_behavior=ee.enum.switches.breakerBehavior.zeroCrossingEnable  i_th=1e-8 A
  Data Type Conversion : DataTypeConversion  OutDataTypeStr=double  SaturateOnIntegerOverflow=off  RndMeth=Floor
  NOT : Logic  Operator=NOT  IconShape=distinctive  AllPortsSameDT=off  OutDataTypeStr=boolean
  Simulink-PS Converter : nesl_utility/Simulink-PS Converter  PhysicalDomain=network_engine_domain  SubClassName=ps_input  LeftPortType=input  RightPortType=output  PseudoPeriodic=off  Frequencies=[]  NoiseDistribution=none  NoiseParameters=[]  Unit=1  AffineConversion=off  FilteringAndDerivatives=provide  SimscapeFilterOrder=1  InputFilterTimeConstant=0.001  UdotUserProvided=0
  Step : Step  Time=1e-6  InitialValue=Three_PhaseBreaker_class('open',1000000,Inf,[0.0166666666666667 0.0833333333333333],'on').objParamMappingDerived.NewDerivedParam.StepInitialValue  FinalValue=0  SampleTime=0
  A : PMIOPort  Side=Left
  B : PMIOPort  Port=2  Side=Left
  C : PMIOPort  Port=3  Side=Left
  a : PMIOPort  Port=4  Side=Right
  b : PMIOPort  Port=5  Side=Right
  c : PMIOPort  Port=6  Side=Right
  wires:
  com/1 -> Add/1
  Add/1 -> NOT/1
  Step/1 -> Add/2
  Data Type Conversion/1 -> Simulink-PS Converter/1
  NOT/1 -> Data Type Conversion/1
  connections:
  Circuit Breaker/LConn1 -- Simulink-PS Converter/RConn1
  c/RConn1 -- Circuit Breaker/RConn3
  b/RConn1 -- Circuit Breaker/RConn2
  a/RConn1 -- Circuit Breaker/RConn1
  Circuit Breaker/LConn4 -- C/RConn1
  Circuit Breaker/LConn3 -- B/RConn1
  Circuit Breaker/LConn2 -- A/RConn1

== system IEEE33_TR_TEMPORAL_RECOGNIZABILITY_MASTER/Bus_2/VI Recorder5 ==
  Vrec : Inport
  Irec : Inport  Port=2
  tag scope: I1to2=global, V1to2=global
  wires:
  Vrec/1 -> [V1to2]
  Irec/1 -> [I1to2]

== system IEEE33_TR_TEMPORAL_RECOGNIZABILITY_MASTER/Bus_20/Bus Load 20 ==
  Electrical Reference : fl_lib/Electrical/Electrical Elements/Electrical Reference
  Wye-Connected Load : ee_lib/Passive/RLC Assemblies/Wye-Connected Load  port_option=ee.enum.threePhasePort.expanded  parameterization=2  component_structure=4  component_structure_PQ=4  R=1 Ohm  L=0.001 H  C=1e-6 F  VRated=12570.4811 V  FRated=60 Hz  P=90000 W  Qpos=40000 V*A  Qneg=Three_PhaseSeriesRLCLoad_class(0).objParamMappingDerived.NewDerivedParam.Qneg V*A  R_parasitic=1e-6 Ohm  G_parasitic=1e-6 1/Ohm  R_parasitic_PQ=1e-6 Ohm  G_parasitic_PQ=1e-6 1/Ohm  Vmag0=12570.4811 V  Vang0=0 deg  Freq0=60 Hz  IL_specify=on  IL_priority=High  IL=[ 0 0 0 ] A  IL_nominal_specify=off  IL_nominal_value=1  IL_nominal_unit=A  VC_specify=on  VC_priority=High  VC=[ 0 0 0 ] V  VC_nominal_specify=off  VC_nominal_value=1  VC_nominal_unit=V
  A : PMIOPort  Side=Left
  B : PMIOPort  Port=2  Side=Left
  C : PMIOPort  Port=3  Side=Left
  connections:
  Electrical Reference/LConn1 -- Wye-Connected Load/RConn1
  Wye-Connected Load/LConn3 -- C/RConn1
  Wye-Connected Load/LConn1 -- A/RConn1
  Wye-Connected Load/LConn2 -- B/RConn1

== system IEEE33_TR_TEMPORAL_RECOGNIZABILITY_MASTER/Bus_20/Bus_20 ==
  Current and Voltage Sensor (Three-Phase) : ee_lib/Sensors & Transducers/Current and Voltage Sensor (Three-Phase)  port_option=ee.enum.threePhasePort.expanded  vMeasurementType=1  outputUnit=2  SRated=100000000 V*A  VRated=500000 V  I_specify=off  I_priority=None  I=[ 0 0 0 ] A  I_nominal_specify=off  I_nominal_value=1  I_nominal_unit=A  V_specify=off  V_priority=None  V=[ 0 0 0 ] V  V_nominal_specify=off  V_nominal_value=1  V_nominal_unit=V
  Igain : Gain  Gain=Three_PhaseV_IMeasuremen_class('phase-to-phase','yes','off','off','off',100000000,500000).objParamMappingDerived.NewDerivedParam.IG
  PS-Simulink Converter : nesl_utility/PS-Simulink Converter  PhysicalDomain=network_engine_domain  SubClassName=ps_output  LeftPortType=input  RightPortType=output  PseudoPeriodic=off  Frequencies=[]  VectorFormat=1-D array  Unit=1  AffineConversion=off
  PS-Simulink Converter1 : nesl_utility/PS-Simulink Converter  PhysicalDomain=network_engine_domain  SubClassName=ps_output  LeftPortType=input  RightPortType=output  PseudoPeriodic=off  Frequencies=[]  VectorFormat=1-D array  Unit=1  AffineConversion=off
  Vgain : Gain  Gain=Three_PhaseV_IMeasuremen_class('phase-to-phase','yes','off','off','off',100000000,500000).objParamMappingDerived.NewDerivedParam.VG
  A : PMIOPort  Side=Left
  B : PMIOPort  Port=2  Side=Left
  C : PMIOPort  Port=3  Side=Left
  a : PMIOPort  Port=4  Side=Right
  b : PMIOPort  Port=5  Side=Right
  c : PMIOPort  Port=6  Side=Right
  Vabc : Outport  VectorParamsAs1DForOutWhenUnconnected=off
  Iabc : Outport  Port=2  VectorParamsAs1DForOutWhenUnconnected=off
  wires:
  Igain/1 -> Iabc/1
  Vgain/1 -> Vabc/1
  PS-Simulink Converter1/1 -> Igain/1
  PS-Simulink Converter/1 -> Vgain/1
  connections:
  Current and Voltage Sensor (Three-Phase)/RConn1 -- PS-Simulink Converter/LConn1
  Current and Voltage Sensor (Three-Phase)/RConn2 -- PS-Simulink Converter1/LConn1
  Current and Voltage Sensor (Three-Phase)/RConn5 -- c/RConn1
  Current and Voltage Sensor (Three-Phase)/RConn4 -- b/RConn1
  Current and Voltage Sensor (Three-Phase)/RConn3 -- a/RConn1
  Current and Voltage Sensor (Three-Phase)/LConn3 -- C/RConn1
  Current and Voltage Sensor (Three-Phase)/LConn1 -- A/RConn1
  Current and Voltage Sensor (Three-Phase)/LConn2 -- B/RConn1

== system IEEE33_TR_TEMPORAL_RECOGNIZABILITY_MASTER/Bus_20/CB3-2 ==
  com : Inport
  Add : Sum
  Circuit Breaker : ee_lib/Switches & Breakers/Circuit Breaker (Three-Phase)  port_option=ee.enum.threePhasePort.expanded  control_port_option=ee.enum.controlport.ps  R_closed=0.01 Ohm  G_open=Three_PhaseBreaker_class('open',1000000,Inf,[0.0166666666666667 0.0833333333333333],'on').objParamMappingDerived.NewDerivedParam.G_open 1/Ohm  threshold=0.5 V  breaker_behavior=ee.enum.switches.breakerBehavior.zeroCrossingEnable  i_th=1e-8 A
  Data Type Conversion : DataTypeConversion  OutDataTypeStr=double  SaturateOnIntegerOverflow=off  RndMeth=Floor
  NOT : Logic  Operator=NOT  IconShape=distinctive  AllPortsSameDT=off  OutDataTypeStr=boolean
  Simulink-PS Converter : nesl_utility/Simulink-PS Converter  PhysicalDomain=network_engine_domain  SubClassName=ps_input  LeftPortType=input  RightPortType=output  PseudoPeriodic=off  Frequencies=[]  NoiseDistribution=none  NoiseParameters=[]  Unit=1  AffineConversion=off  FilteringAndDerivatives=provide  SimscapeFilterOrder=1  InputFilterTimeConstant=0.001  UdotUserProvided=0
  Step : Step  Time=1e-6  InitialValue=Three_PhaseBreaker_class('open',1000000,Inf,[0.0166666666666667 0.0833333333333333],'on').objParamMappingDerived.NewDerivedParam.StepInitialValue  FinalValue=0  SampleTime=0
  A : PMIOPort  Side=Left
  B : PMIOPort  Port=2  Side=Left
  C : PMIOPort  Port=3  Side=Left
  a : PMIOPort  Port=4  Side=Right
  b : PMIOPort  Port=5  Side=Right
  c : PMIOPort  Port=6  Side=Right
  wires:
  com/1 -> Add/1
  Add/1 -> NOT/1
  Step/1 -> Add/2
  Data Type Conversion/1 -> Simulink-PS Converter/1
  NOT/1 -> Data Type Conversion/1
  connections:
  Circuit Breaker/LConn1 -- Simulink-PS Converter/RConn1
  c/RConn1 -- Circuit Breaker/RConn3
  b/RConn1 -- Circuit Breaker/RConn2
  a/RConn1 -- Circuit Breaker/RConn1
  Circuit Breaker/LConn4 -- C/RConn1
  Circuit Breaker/LConn3 -- B/RConn1
  Circuit Breaker/LConn2 -- A/RConn1

== system IEEE33_TR_TEMPORAL_RECOGNIZABILITY_MASTER/Bus_20/VI Recorder1 ==
  Vrec : Inport
  Irec : Inport  Port=2
  tag scope: I19to20=global, V19to20=global
  wires:
  Vrec/1 -> [V19to20]
  Irec/1 -> [I19to20]

== system IEEE33_TR_TEMPORAL_RECOGNIZABILITY_MASTER/Bus_21/Bus Load 21 ==
  Electrical Reference : fl_lib/Electrical/Electrical Elements/Electrical Reference
  Wye-Connected Load : ee_lib/Passive/RLC Assemblies/Wye-Connected Load  port_option=ee.enum.threePhasePort.expanded  parameterization=2  component_structure=4  component_structure_PQ=4  R=1 Ohm  L=0.001 H  C=1e-6 F  VRated=12561.5558 V  FRated=60 Hz  P=90000 W  Qpos=40000 V*A  Qneg=Three_PhaseSeriesRLCLoad_class(0).objParamMappingDerived.NewDerivedParam.Qneg V*A  R_parasitic=1e-6 Ohm  G_parasitic=1e-6 1/Ohm  R_parasitic_PQ=1e-6 Ohm  G_parasitic_PQ=1e-6 1/Ohm  Vmag0=12561.5558 V  Vang0=0 deg  Freq0=60 Hz  IL_specify=on  IL_priority=High  IL=[ 0 0 0 ] A  IL_nominal_specify=off  IL_nominal_value=1  IL_nominal_unit=A  VC_specify=on  VC_priority=High  VC=[ 0 0 0 ] V  VC_nominal_specify=off  VC_nominal_value=1  VC_nominal_unit=V
  A : PMIOPort  Side=Left
  B : PMIOPort  Port=2  Side=Left
  C : PMIOPort  Port=3  Side=Left
  connections:
  Electrical Reference/LConn1 -- Wye-Connected Load/RConn1
  Wye-Connected Load/LConn3 -- C/RConn1
  Wye-Connected Load/LConn1 -- A/RConn1
  Wye-Connected Load/LConn2 -- B/RConn1

== system IEEE33_TR_TEMPORAL_RECOGNIZABILITY_MASTER/Bus_21/Bus_21 ==
  Current and Voltage Sensor (Three-Phase) : ee_lib/Sensors & Transducers/Current and Voltage Sensor (Three-Phase)  port_option=ee.enum.threePhasePort.expanded  vMeasurementType=1  outputUnit=2  SRated=100000000 V*A  VRated=500000 V  I_specify=off  I_priority=None  I=[ 0 0 0 ] A  I_nominal_specify=off  I_nominal_value=1  I_nominal_unit=A  V_specify=off  V_priority=None  V=[ 0 0 0 ] V  V_nominal_specify=off  V_nominal_value=1  V_nominal_unit=V
  Igain : Gain  Gain=Three_PhaseV_IMeasuremen_class('phase-to-phase','yes','off','off','off',100000000,500000).objParamMappingDerived.NewDerivedParam.IG
  PS-Simulink Converter : nesl_utility/PS-Simulink Converter  PhysicalDomain=network_engine_domain  SubClassName=ps_output  LeftPortType=input  RightPortType=output  PseudoPeriodic=off  Frequencies=[]  VectorFormat=1-D array  Unit=1  AffineConversion=off
  PS-Simulink Converter1 : nesl_utility/PS-Simulink Converter  PhysicalDomain=network_engine_domain  SubClassName=ps_output  LeftPortType=input  RightPortType=output  PseudoPeriodic=off  Frequencies=[]  VectorFormat=1-D array  Unit=1  AffineConversion=off
  Vgain : Gain  Gain=Three_PhaseV_IMeasuremen_class('phase-to-phase','yes','off','off','off',100000000,500000).objParamMappingDerived.NewDerivedParam.VG
  A : PMIOPort  Side=Left
  B : PMIOPort  Port=2  Side=Left
  C : PMIOPort  Port=3  Side=Left
  a : PMIOPort  Port=4  Side=Right
  b : PMIOPort  Port=5  Side=Right
  c : PMIOPort  Port=6  Side=Right
  Vabc : Outport  VectorParamsAs1DForOutWhenUnconnected=off
  Iabc : Outport  Port=2  VectorParamsAs1DForOutWhenUnconnected=off
  wires:
  Igain/1 -> Iabc/1
  Vgain/1 -> Vabc/1
  PS-Simulink Converter1/1 -> Igain/1
  PS-Simulink Converter/1 -> Vgain/1
  connections:
  Current and Voltage Sensor (Three-Phase)/RConn1 -- PS-Simulink Converter/LConn1
  Current and Voltage Sensor (Three-Phase)/RConn2 -- PS-Simulink Converter1/LConn1
  Current and Voltage Sensor (Three-Phase)/RConn5 -- c/RConn1
  Current and Voltage Sensor (Three-Phase)/RConn4 -- b/RConn1
  Current and Voltage Sensor (Three-Phase)/RConn3 -- a/RConn1
  Current and Voltage Sensor (Three-Phase)/LConn3 -- C/RConn1
  Current and Voltage Sensor (Three-Phase)/LConn1 -- A/RConn1
  Current and Voltage Sensor (Three-Phase)/LConn2 -- B/RConn1

== system IEEE33_TR_TEMPORAL_RECOGNIZABILITY_MASTER/Bus_21/CB3-1 ==
  com : Inport
  Add : Sum
  Circuit Breaker : ee_lib/Switches & Breakers/Circuit Breaker (Three-Phase)  port_option=ee.enum.threePhasePort.expanded  control_port_option=ee.enum.controlport.ps  R_closed=0.01 Ohm  G_open=Three_PhaseBreaker_class('open',1000000,Inf,[0.0166666666666667 0.0833333333333333],'on').objParamMappingDerived.NewDerivedParam.G_open 1/Ohm  threshold=0.5 V  breaker_behavior=ee.enum.switches.breakerBehavior.zeroCrossingEnable  i_th=1e-8 A
  Data Type Conversion : DataTypeConversion  OutDataTypeStr=double  SaturateOnIntegerOverflow=off  RndMeth=Floor
  NOT : Logic  Operator=NOT  IconShape=distinctive  AllPortsSameDT=off  OutDataTypeStr=boolean
  Simulink-PS Converter : nesl_utility/Simulink-PS Converter  PhysicalDomain=network_engine_domain  SubClassName=ps_input  LeftPortType=input  RightPortType=output  PseudoPeriodic=off  Frequencies=[]  NoiseDistribution=none  NoiseParameters=[]  Unit=1  AffineConversion=off  FilteringAndDerivatives=provide  SimscapeFilterOrder=1  InputFilterTimeConstant=0.001  UdotUserProvided=0
  Step : Step  Time=1e-6  InitialValue=Three_PhaseBreaker_class('open',1000000,Inf,[0.0166666666666667 0.0833333333333333],'on').objParamMappingDerived.NewDerivedParam.StepInitialValue  FinalValue=0  SampleTime=0
  A : PMIOPort  Side=Left
  B : PMIOPort  Port=2  Side=Left
  C : PMIOPort  Port=3  Side=Left
  a : PMIOPort  Port=4  Side=Right
  b : PMIOPort  Port=5  Side=Right
  c : PMIOPort  Port=6  Side=Right
  wires:
  com/1 -> Add/1
  Add/1 -> NOT/1
  Step/1 -> Add/2
  Data Type Conversion/1 -> Simulink-PS Converter/1
  NOT/1 -> Data Type Conversion/1
  connections:
  Circuit Breaker/LConn1 -- Simulink-PS Converter/RConn1
  c/RConn1 -- Circuit Breaker/RConn3
  b/RConn1 -- Circuit Breaker/RConn2
  a/RConn1 -- Circuit Breaker/RConn1
  Circuit Breaker/LConn4 -- C/RConn1
  Circuit Breaker/LConn3 -- B/RConn1
  Circuit Breaker/LConn2 -- A/RConn1

== system IEEE33_TR_TEMPORAL_RECOGNIZABILITY_MASTER/Bus_21/CB3-2 ==
  com : Inport
  Add : Sum
  Circuit Breaker : ee_lib/Switches & Breakers/Circuit Breaker (Three-Phase)  port_option=ee.enum.threePhasePort.expanded  control_port_option=ee.enum.controlport.ps  R_closed=0.01 Ohm  G_open=Three_PhaseBreaker_class('open',1000000,Inf,[0.0166666666666667 0.0833333333333333],'on').objParamMappingDerived.NewDerivedParam.G_open 1/Ohm  threshold=0.5 V  breaker_behavior=ee.enum.switches.breakerBehavior.zeroCrossingEnable  i_th=1e-8 A
  Data Type Conversion : DataTypeConversion  OutDataTypeStr=double  SaturateOnIntegerOverflow=off  RndMeth=Floor
  NOT : Logic  Operator=NOT  IconShape=distinctive  AllPortsSameDT=off  OutDataTypeStr=boolean
  Simulink-PS Converter : nesl_utility/Simulink-PS Converter  PhysicalDomain=network_engine_domain  SubClassName=ps_input  LeftPortType=input  RightPortType=output  PseudoPeriodic=off  Frequencies=[]  NoiseDistribution=none  NoiseParameters=[]  Unit=1  AffineConversion=off  FilteringAndDerivatives=provide  SimscapeFilterOrder=1  InputFilterTimeConstant=0.001  UdotUserProvided=0
  Step : Step  Time=1e-6  InitialValue=Three_PhaseBreaker_class('open',1000000,Inf,[0.0166666666666667 0.0833333333333333],'on').objParamMappingDerived.NewDerivedParam.StepInitialValue  FinalValue=0  SampleTime=0
  A : PMIOPort  Side=Left
  B : PMIOPort  Port=2  Side=Left
  C : PMIOPort  Port=3  Side=Left
  a : PMIOPort  Port=4  Side=Right
  b : PMIOPort  Port=5  Side=Right
  c : PMIOPort  Port=6  Side=Right
  wires:
  com/1 -> Add/1
  Add/1 -> NOT/1
  Step/1 -> Add/2
  Data Type Conversion/1 -> Simulink-PS Converter/1
  NOT/1 -> Data Type Conversion/1
  connections:
  Circuit Breaker/LConn1 -- Simulink-PS Converter/RConn1
  c/RConn1 -- Circuit Breaker/RConn3
  b/RConn1 -- Circuit Breaker/RConn2
  a/RConn1 -- Circuit Breaker/RConn1
  Circuit Breaker/LConn4 -- C/RConn1
  Circuit Breaker/LConn3 -- B/RConn1
  Circuit Breaker/LConn2 -- A/RConn1

== system IEEE33_TR_TEMPORAL_RECOGNIZABILITY_MASTER/Bus_21/VI Recorder2 ==
  Vrec : Inport
  Irec : Inport  Port=2
  tag scope: I20to21=global, V20to21=global
  wires:
  Vrec/1 -> [V20to21]
  Irec/1 -> [I20to21]

== system IEEE33_TR_TEMPORAL_RECOGNIZABILITY_MASTER/Bus_22/Bus Load 22 ==
  Electrical Reference : fl_lib/Electrical/Electrical Elements/Electrical Reference
  Wye-Connected Load : ee_lib/Passive/RLC Assemblies/Wye-Connected Load  port_option=ee.enum.threePhasePort.expanded  parameterization=2  component_structure=4  component_structure_PQ=4  R=1 Ohm  L=0.001 H  C=1e-6 F  VRated=12553.4914 V  FRated=60 Hz  P=90000 W  Qpos=40000 V*A  Qneg=Three_PhaseSeriesRLCLoad_class(0).objParamMappingDerived.NewDerivedParam.Qneg V*A  R_parasitic=1e-6 Ohm  G_parasitic=1e-6 1/Ohm  R_parasitic_PQ=1e-6 Ohm  G_parasitic_PQ=1e-6 1/Ohm  Vmag0=12553.4914 V  Vang0=0 deg  Freq0=60 Hz  IL_specify=on  IL_priority=High  IL=[ 0 0 0 ] A  IL_nominal_specify=off  IL_nominal_value=1  IL_nominal_unit=A  VC_specify=on  VC_priority=High  VC=[ 0 0 0 ] V  VC_nominal_specify=off  VC_nominal_value=1  VC_nominal_unit=V
  A : PMIOPort  Side=Left
  B : PMIOPort  Port=2  Side=Left
  C : PMIOPort  Port=3  Side=Left
  connections:
  Electrical Reference/LConn1 -- Wye-Connected Load/RConn1
  Wye-Connected Load/LConn3 -- C/RConn1
  Wye-Connected Load/LConn1 -- A/RConn1
  Wye-Connected Load/LConn2 -- B/RConn1
